simulink model "simulink_modal"  (R2025b)
settings: Solver=VariableStepAuto  StartTime=0.0  StopTime=10.0  RelTol=1e-3
values from neighbouring files (symbols this model uses):
  g = 9.80665    [init_pendulum.m]
  pin1_angle_rad = deg2rad(pin1_angle)    [init_pendulum.m]
  pin2_angle_rad = deg2rad(pin2_angle)    [init_pendulum.m]
  rod1_Innertia = 0.25 * rod1_mass * (rod1_radius^2) + (1/12) * rod1_mass * (rod1_length^2)    (= 1.78039946165)    [init_pendulum.m]
  rod1_length = 1    [init_pendulum.m]
  rod1_mass = density1*(pi*rod1_radius^2*rod1_length)    (= 21.2057504117)    [init_pendulum.m]
  rod2_Innertia = 0.25 * rod2_mass * (rod2_radius^2) + (1/12) * rod2_mass * (rod2_length^2)    (= 2.15444533697)    [init_pendulum.m]
  rod2_length = 0.75    [init_pendulum.m]
  rod2_mass = density2*(pi*rod2_radius^2*rod2_length)    (= 45.3567439362)    [init_pendulum.m]
settings Model: Creator=Hp  LastModifiedBy=Hp

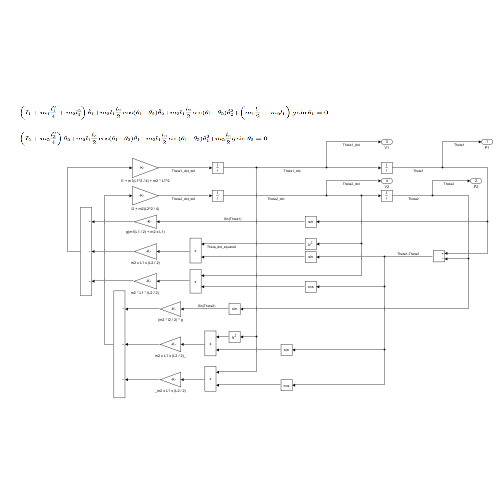
[thumbnail: Simulink's stored preview of the top-level diagram]
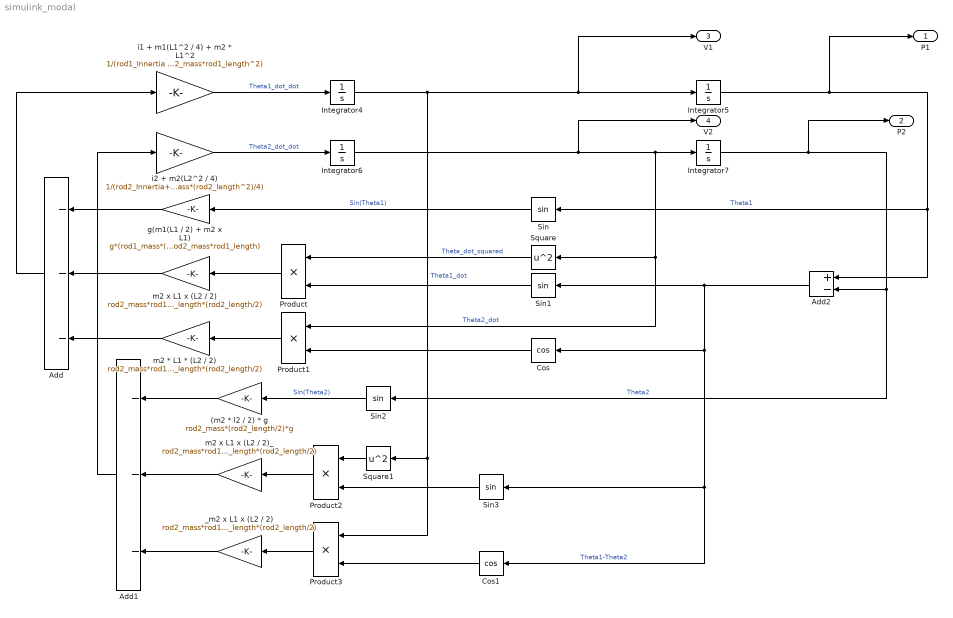
== system simulink_modal ==
  (m2 * l2 / 2) * g : Gain  Gain=rod2_mass*(rod2_length/2)*g
  Add : Sum  Inputs=---
  Add1 : Sum  Inputs=---
  Add2 : Sum  Inputs=+-
  Cos : Trigonometry  Operator=cos
  Cos1 : Trigonometry  Operator=cos
  Integrator4 : Integrator
  Integrator5 : Integrator  InitialCondition=pin1_angle_rad
  Integrator6 : Integrator
  Integrator7 : Integrator  InitialCondition=pin2_angle_rad
  Product{,1..3} (4 alike) : Product
  Sin{,1..3} (4 alike) : Trigonometry
  Square : Math  Operator=square
  Square1 : Math  Operator=square
  _m2 x L1 x (L2 / 2) : Gain  Gain=rod2_mass*rod1_length*(rod2_length/2)
  g(m1(L1 / 2) + m2 x L1) : Gain  Gain=g*(rod1_mass*(rod1_length/2) + rod2_mass*rod1_length)
  i1 + m1(L1^2 / 4) + m2 * L1^2 : Gain  Gain=1/(rod1_Innertia + rod1_mass*(rod1_length^2/4) + rod2_mass*rod1_length^2)
  i2 + m2(L2^2 / 4) : Gain  Gain=1/(rod2_Innertia+rod2_mass*(rod2_length^2)/4)
  "m2 * L1 * (L2 / 2) " : Gain  Gain=rod2_mass*rod1_length*(rod2_length/2)
  m2 x L1 x (L2 / 2) : Gain  Gain=rod2_mass*rod1_length*(rod2_length/2)
  m2 x L1 x (L2 / 2)_ : Gain  Gain=rod2_mass*rod1_length*(rod2_length/2)
  P1 : Outport
  P2 : Outport  Port=2
  V1 : Outport  Port=3
  V2 : Outport  Port=4
  wires:
  Product1/1 -> "m2 * L1 * (L2 / 2) "/1
  Cos/1 -> Product1/2
  Product2/1 -> m2 x L1 x (L2 / 2)_/1
  _m2 x L1 x (L2 / 2)/1 -> Add1/3
  Integrator4/1 -> Product3/1, Square1/1, V1/1, Integrator5/1  "Theta1_dot"
  m2 x L1 x (L2 / 2)/1 -> Add/2
  Add/1 -> i1 + m1(L1^2 / 4) + m2 * L1^2/1
  Cos1/1 -> Product3/2
  i2 + m2(L2^2 / 4)/1 -> Integrator6/1  "Theta2_dot_dot"
  Sin1/1 -> Product/2
  Add2/1 -> Cos1/1, Sin3/1, Cos/1, Sin1/1  "Theta1-Theta2"
  Square1/1 -> Product2/1
  Sin/1 -> g(m1(L1 / 2) + m2 x L1)/1  "Sin(Theta1)"
  Sin2/1 -> (m2 * l2 / 2) * g/1  "Sin(Theta2)"
  Integrator7/1 -> P2/1, Add2/2, Sin2/1  "Theta2"
  "m2 * L1 * (L2 / 2) "/1 -> Add/3
  Add1/1 -> i2 + m2(L2^2 / 4)/1
  i1 + m1(L1^2 / 4) + m2 * L1^2/1 -> Integrator4/1  "Theta1_dot_dot"
  Square/1 -> Product/1  "Theta_dot_squared"
  m2 x L1 x (L2 / 2)_/1 -> Add1/2
  Product/1 -> m2 x L1 x (L2 / 2)/1
  Integrator5/1 -> P1/1, Add2/1, Sin/1  "Thete1"
  Integrator6/1 -> V2/1, Integrator7/1, Product1/1, Square/1  "Theta2_dot"
  g(m1(L1 / 2) + m2 x L1)/1 -> Add/1
  Sin3/1 -> Product2/2
  (m2 * l2 / 2) * g/1 -> Add1/1
  Product3/1 -> _m2 x L1 x (L2 / 2)/1
